simulink model "LTI_aumentado_vs_Modelo_NL"  (R2026a)
settings: Solver=VariableStepAuto  StopTime=5
undefined symbols (not defined in the file): alpha_Cu, b_eq, C_ts, g, J_eq_min, k_l, L_d, L_ls, L_q, lambda, magnitude, Pp, r_m2l, R_sREF, R_tsamb, T_sREF
settings Model: Creator=lamun  LastModifiedBy=lamun

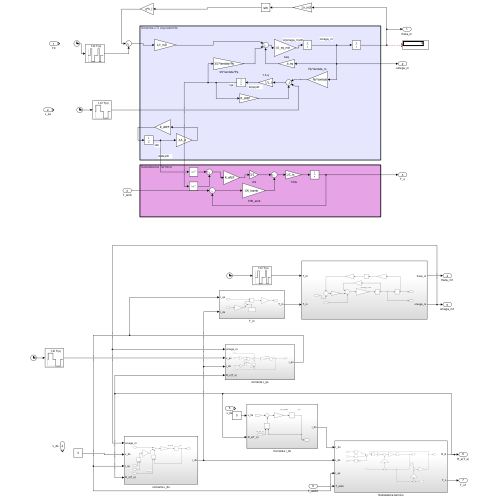
[thumbnail: Simulink's stored preview of the top-level diagram]
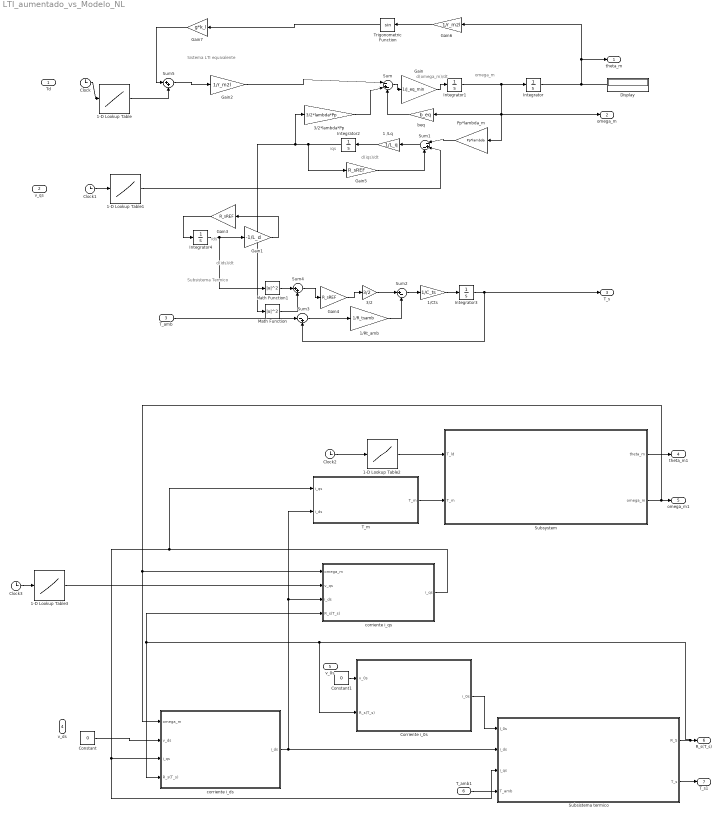
== system LTI_aumentado_vs_Modelo_NL ==
  note: Sistema LTI equivalente
  note: d(omega_m)/dt
  note: d(ids)/dt
  note: d(iqs)/dt
  note: iqs
  note: omega_m
  note: ids
  note: Subsistema Termico
  Td : Inport
  v_qs : Inport  Port=2
  T_amb : Inport  Port=3
  v_ds : Inport  Port=4
  v_0s : Inport  Port=5
  T_amb1 : Inport  Port=6
  1 /Lq : Gain  Gain=1/L_q
  1-D Lookup Table : Lookup_n-D  NumberOfTableDimensions=1  BreakpointsForDimension1=[0.0, 0.1, 0.101, 0.3, 0.301, 0.5, 0.501, 0.7, 0.701, 0.9, 0.901, 1.1, 1.101, 1.3, 1.301, 1.5, 1.501, 1.7, 1.701, 1.9, 1.901, 2.0]  Table=[0.0, 0.0, 0.0, 0.0, 6.28, 6.28, -6.28, -6.28, -6.28, -6.28, 0.0, 0.0, 0.0, 0.0, 6.28, 6.28, -6.28, -6.28, 0.0, 0.0, 0.0, 0.0]  InternalRulePriority=Speed  RndMeth=Simplest
  1-D Lookup Table1 : Lookup_n-D  NumberOfTableDimensions=1  BreakpointsForDimension1=[0.0, 0.1, 0.101, 0.3, 0.301, 0.5, 0.501, 0.7, 0.701, 0.9, 0.901, 1.1, 1.101, 1.3, 1.301, 1.5, 1.501, 1.7, 1.701, 1.9, 1.901, 2.0]  Table=[0.0, 0.0, 19.596, 19.596, 19.596, 19.596, 19.596, 19.596, 0.0, 0.0, 0.0, 0.0, -19.596, -19.596, -19.596, -19.596, -19.596, -19.596, 0.0, 0.0, 0.0, 0.0]  InternalRulePriority=Speed  RndMeth=Simplest
  1-D Lookup Table2 : Lookup_n-D  NumberOfTableDimensions=1  BreakpointsForDimension1=[0.0, 0.1, 0.101, 0.3, 0.301, 0.5, 0.501, 0.7, 0.701, 0.9, 0.901, 1.1, 1.101, 1.3, 1.301, 1.5, 1.501, 1.7, 1.701, 1.9, 1.901, 2.0]  Table=[0.0, 0.0, 0.0, 0.0, 6.28, 6.28, -6.28, -6.28, -6.28, -6.28, 0.0, 0.0, 0.0, 0.0, 6.28, 6.28, -6.28, -6.28, 0.0, 0.0, 0.0, 0.0]  InternalRulePriority=Speed  RndMeth=Simplest
  1-D Lookup Table3 : Lookup_n-D  NumberOfTableDimensions=1  BreakpointsForDimension1=[0.0, 0.1, 0.101, 0.3, 0.301, 0.5, 0.501, 0.7, 0.701, 0.9, 0.901, 1.1, 1.101, 1.3, 1.301, 1.5, 1.501, 1.7, 1.701, 1.9, 1.901, 2.0]  Table=[0.0, 0.0, 19.596, 19.596, 19.596, 19.596, 19.596, 19.596, 0.0, 0.0, 0.0, 0.0, -19.596, -19.596, -19.596, -19.596, -19.596, -19.596, 0.0, 0.0, 0.0, 0.0]  InternalRulePriority=Speed  RndMeth=Simplest
  1/Cts : Gain  Gain=1/C_ts
  1/Rt_amb : Gain  Gain=1/R_tsamb
  3/2 : Gain  Gain=3/2
  3/2*lambda*Pp : Gain  Gain=3/2*lambda*Pp
  Clock{,1..3} (4 alike) : Clock
  Constant : Constant  Value=0
  Constant1 : Constant  Value=0
  Corriente i_0s : Subsystem
  Display : Display
  Gain : Gain  Gain=1/J_eq_min
  Gain1 : Gain  Gain=-1/L_d
  Gain2 : Gain  Gain=1/r_m2l
  Gain3 : Gain  Gain=R_sREF
  Gain4 : Gain  Gain=R_sREF
  Gain5 : Gain  Gain=R_sREF
  Gain6 : Gain  Gain=1/r_m2l
  Gain7 : Gain  Gain=g*k_l
  Integrator{,1..4} (5 alike) : Integrator
  Math Function : Math  Operator=magnitude^2
  Math Function1 : Math  Operator=magnitude^2
  Pp*lambda_m : Gain  Gain=Pp*lambda
  Subsistema termico : Subsystem
  Subsystem : Subsystem
  Sum : Sum  Inputs=|-+-
  Sum1 : Sum  Inputs=|-+-
  Sum2 : Sum  Inputs=|+-
  Sum3 : Sum  Inputs=|-+
  Sum4 : Sum  Inputs=|++
  Sum5 : Sum  Inputs=|++
  T_m : Subsystem
  Trigonometric Function : Trigonometry
  beq : Gain  Gain=b_eq
  corriente i_ds : Subsystem
  corriente i_qs : Subsystem
  theta_m : Outport
  omega_m : Outport  Port=2
  T_s : Outport  Port=3
  theta_m1 : Outport  Port=4
  omega_m1 : Outport  Port=5
  R_s(T_s) : Outport  Port=6
  T_s1 : Outport  Port=7
  wires:
  Gain2/1 -> Sum/1
  Clock/1 -> 1-D Lookup Table/1
  1-D Lookup Table1/1 -> Sum1/2
  T_amb/1 -> Sum3/1
  Gain4/1 -> 3/2/1
  1-D Lookup Table/1 -> Sum5/2
  Sum2/1 -> 1/Cts/1
  1/Rt_amb/1 -> Sum2/2
  1 /Lq/1 -> Integrator2/1
  Math Function1/1 -> Sum4/1
  Sum4/1 -> Gain4/1
  Integrator3/1 -> T_s/1, Sum3/2
  beq/1 -> Sum/3
  3/2/1 -> Sum2/1
  Math Function/1 -> Sum4/2
  Clock1/1 -> 1-D Lookup Table1/1
  Integrator2/1 -> Gain5/1, 3/2*lambda*Pp/1, Math Function/1
  Sum/1 -> Gain/1
  Integrator/1 -> Gain6/1, theta_m/1
  Gain/1 -> Integrator1/1
  Sum3/1 -> 1/Rt_amb/1
  Integrator4/1 -> Gain1/1, Math Function1/1
  Integrator1/1 -> Integrator/1, beq/1, omega_m/1, Pp*lambda_m/1
  Gain1/1 -> Gain3/1
  Pp*lambda_m/1 -> Sum1/1
  Sum1/1 -> 1 /Lq/1
  3/2*lambda*Pp/1 -> Sum/2
  1/Cts/1 -> Integrator3/1
  Gain3/1 -> Integrator4/1
  Gain5/1 -> Sum1/3
  Sum5/1 -> Gain2/1
  Gain6/1 -> Trigonometric Function/1
  Trigonometric Function/1 -> Gain7/1
  Gain7/1 -> Sum5/1
  1-D Lookup Table3/1 -> corriente i_qs/2(v_qs)
  corriente i_qs/1(i_qs) -> Subsistema termico/3(i_qs), corriente i_ds/3(i_qs), T_m/1(i_qs)
  Subsystem/2(omega_m) -> corriente i_ds/1(omega_m), corriente i_qs/1(omega_m), omega_m1/1
  T_m/1(T_m) -> Subsystem/2(T_m)
  1-D Lookup Table2/1 -> Subsystem/1(T_ld)
  Subsystem/1(theta_m) -> theta_m1/1
  Clock2/1 -> 1-D Lookup Table2/1
  Clock3/1 -> 1-D Lookup Table3/1
  corriente i_ds/1(i_ds) -> Subsistema termico/2(i_ds), T_m/2(i_ds), corriente i_qs/3(i_ds)
  Subsistema termico/1(R_S) -> corriente i_qs/4(R_s(T_s)), corriente i_ds/4(R_s(T_s)), Corriente i_0s/2(R_s(T_s)), R_s(T_s)/1
  T_amb1/1 -> Subsistema termico/4(T_amb)
  Subsistema termico/2(T_s) -> T_s1/1
  Corriente i_0s/1(i_0s) -> Subsistema termico/1(I_0s)
  Constant/1 -> corriente i_ds/2(v_ds)
  Constant1/1 -> Corriente i_0s/1(v_0s)

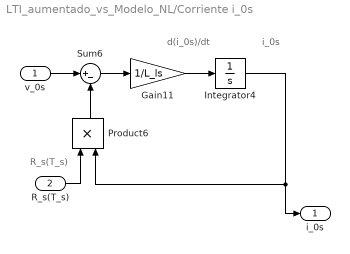
== system LTI_aumentado_vs_Modelo_NL/Corriente i_0s ==
  note: d(i_0s)/dt
  note: R_s(T_s)
  note: i_0s
  v_0s : Inport
  R_s(T_s) : Inport  Port=2
  Gain11 : Gain  Gain=1/L_ls
  Integrator4 : Integrator
  Product6 : Product
  Sum6 : Sum  Inputs=|+-
  i_0s : Outport
  wires:
  v_0s/1 -> Sum6/1
  Integrator4/1 -> i_0s/1, Product6/2
  Sum6/1 -> Gain11/1
  R_s(T_s)/1 -> Product6/1
  Product6/1 -> Sum6/2
  Gain11/1 -> Integrator4/1

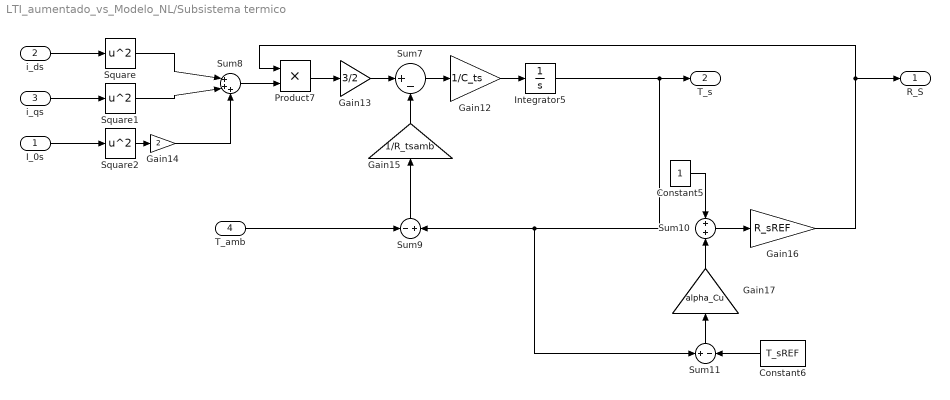
== system LTI_aumentado_vs_Modelo_NL/Subsistema termico ==
  I_0s : Inport
  i_ds : Inport  Port=2
  i_qs : Inport  Port=3
  T_amb : Inport  Port=4
  Constant5 : Constant
  Constant6 : Constant  Value=T_sREF
  Gain12 : Gain  Gain=1/C_ts
  Gain13 : Gain  Gain=3/2
  Gain14 : Gain  Gain=2
  Gain15 : Gain  Gain=1/R_tsamb
  Gain16 : Gain  Gain=R_sREF
  Gain17 : Gain  Gain=alpha_Cu
  Integrator5 : Integrator
  Product7 : Product
  Square : Math  Operator=square
  Square1 : Math  Operator=square
  Square2 : Math  Operator=square
  Sum10 : Sum
  Sum11 : Sum  Inputs=+-
  Sum7 : Sum  Inputs=|+-
  Sum8 : Sum  Inputs=|+++
  Sum9 : Sum  Inputs=-+
  R_S : Outport
  T_s : Outport  Port=2
  wires:
  Constant6/1 -> Sum11/2
  Gain15/1 -> Sum7/2
  Square1/1 -> Sum8/2
  Gain14/1 -> Sum8/3
  Sum9/1 -> Gain15/1
  Square2/1 -> Gain14/1
  i_ds/1 -> Square/1
  Integrator5/1 -> Sum9/2, Sum11/1, T_s/1
  Sum10/1 -> Gain16/1
  Constant5/1 -> Sum10/1
  Gain13/1 -> Sum7/1
  Gain12/1 -> Integrator5/1
  Sum7/1 -> Gain12/1
  Sum8/1 -> Product7/2
  Product7/1 -> Gain13/1
  Square/1 -> Sum8/1
  Sum11/1 -> Gain17/1
  Gain17/1 -> Sum10/2
  T_amb/1 -> Sum9/1
  I_0s/1 -> Square2/1
  i_qs/1 -> Square1/1
  Gain16/1 -> R_S/1, Product7/1

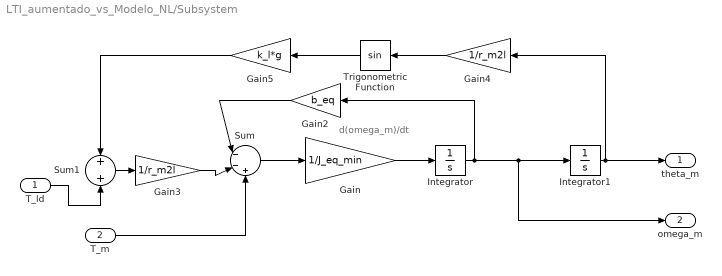
== system LTI_aumentado_vs_Modelo_NL/Subsystem ==
  note: d(omega_m)/dt
  T_ld : Inport
  T_m : Inport  Port=2
  Gain : Gain  Gain=1/J_eq_min
  Gain2 : Gain  Gain=b_eq
  Gain3 : Gain  Gain=1/r_m2l
  Gain4 : Gain  Gain=1/r_m2l
  Gain5 : Gain  Gain=k_l*g
  Integrator : Integrator
  Integrator1 : Integrator
  Sum : Sum  Inputs=|--+
  Sum1 : Sum
  Trigonometric Function : Trigonometry
  theta_m : Outport
  omega_m : Outport  Port=2
  wires:
  Sum/1 -> Gain/1
  Integrator1/1 -> theta_m/1, Gain4/1
  Gain5/1 -> Sum1/1
  Gain4/1 -> Trigonometric Function/1
  Trigonometric Function/1 -> Gain5/1
  Gain/1 -> Integrator/1
  Integrator/1 -> Gain2/1, omega_m/1, Integrator1/1
  Gain2/1 -> Sum/1
  T_ld/1 -> Sum1/2
  T_m/1 -> Sum/3
  Sum1/1 -> Gain3/1
  Gain3/1 -> Sum/2

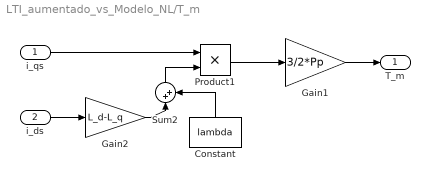
== system LTI_aumentado_vs_Modelo_NL/T_m ==
  i_qs : Inport
  i_ds : Inport  Port=2
  Constant : Constant  Value=lambda
  Gain1 : Gain  Gain=3/2*Pp
  Gain2 : Gain  Gain=L_d-L_q
  Product1 : Product
  Sum2 : Sum  Inputs=|++
  T_m : Outport
  wires:
  Gain2/1 -> Sum2/1
  Constant/1 -> Sum2/2
  i_ds/1 -> Gain2/1
  Product1/1 -> Gain1/1
  Sum2/1 -> Product1/2
  Gain1/1 -> T_m/1
  i_qs/1 -> Product1/1

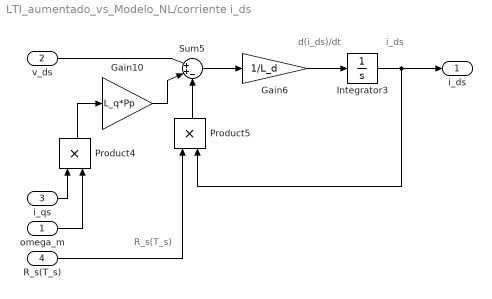
== system LTI_aumentado_vs_Modelo_NL/corriente i_ds ==
  note: d(i_ds)/dt
  note: i_ds
  note: R_s(T_s)
  omega_m : Inport
  v_ds : Inport  Port=2
  i_qs : Inport  Port=3
  R_s(T_s) : Inport  Port=4
  Gain10 : Gain  Gain=L_q*Pp
  Gain6 : Gain  Gain=1/L_d
  Integrator3 : Integrator
  Product4 : Product
  Product5 : Product
  Sum5 : Sum  Inputs=|++-
  i_ds : Outport
  wires:
  i_qs/1 -> Product4/1
  Product5/1 -> Sum5/3
  Gain6/1 -> Integrator3/1
  v_ds/1 -> Sum5/1
  Sum5/1 -> Gain6/1
  Gain10/1 -> Sum5/2
  Product4/1 -> Gain10/1
  omega_m/1 -> Product4/2
  Integrator3/1 -> Product5/2, i_ds/1
  R_s(T_s)/1 -> Product5/1

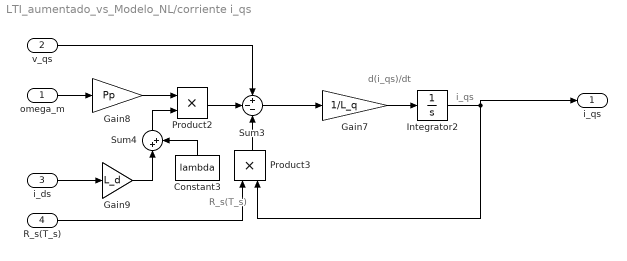
== system LTI_aumentado_vs_Modelo_NL/corriente i_qs ==
  note: d(i_qs)/dt
  note: i_qs
  note: R_s(T_s)
  omega_m : Inport
  v_qs : Inport  Port=2
  i_ds : Inport  Port=3
  R_s(T_s) : Inport  Port=4
  Constant3 : Constant  Value=lambda
  Gain7 : Gain  Gain=1/L_q
  Gain8 : Gain  Gain=Pp
  Gain9 : Gain  Gain=L_d
  Integrator2 : Integrator
  Product2 : Product
  Product3 : Product
  Sum3 : Sum  Inputs=+--
  Sum4 : Sum  Inputs=|++
  i_qs : Outport
  wires:
  Sum3/1 -> Gain7/1
  omega_m/1 -> Gain8/1
  Gain9/1 -> Sum4/1
  Gain7/1 -> Integrator2/1
  Sum4/1 -> Product2/2
  v_qs/1 -> Sum3/1
  Product2/1 -> Sum3/2
  Constant3/1 -> Sum4/2
  Product3/1 -> Sum3/3
  i_ds/1 -> Gain9/1
  Integrator2/1 -> Product3/2, i_qs/1
  R_s(T_s)/1 -> Product3/1
  Gain8/1 -> Product2/1
